simulink model "boost_cycle_R2021b"  (R2021b)
settings: Solver=FixedStepDiscrete  StartTime=0  StopTime=(N-1)*Ts  FixedStep=Ts  RelTol=1e-3
model workspace (MAT data in the model file):
  CP = [2 0.03 20 0 0 1 0 0 0.15 12 12 48 0.5 0.05 0.9 0.0005 5e-05 0 60 0 18 0 15 0 60 24 0 0 0 0 0 0]
  LP = [1 0.05 20 10 0 0 0]
  N = 2000
  PP = [0.0005 0.00047 5e-05 0 0 0 0 100 0 0]
  Ts = 5e-05
  VP = [0 24 0 0 0 0 0]
  X0 = [0; 0; 0; 0; 0; 0.5; 0.5; 0.5]
  XP0 = [0; 24; 24]
settings Model: Creator=runner  LastModifiedBy=runner
settings DebuggingCC: AlgebraicLoopMsg=error  UnconnectedInputMsg=none  UnconnectedOutputMsg=none  UnconnectedLineMsg=none
settings ModelReferenceCC: EnableRefExpFcnMdlSchedulingChecks=off
settings RTWCC: DLArmComputeVersion=20.02.1

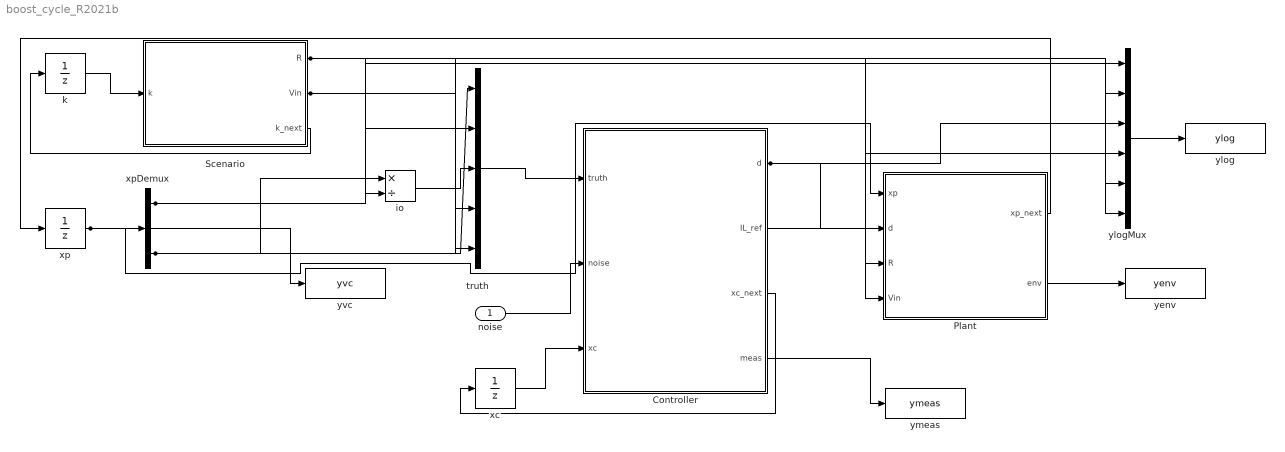
== system boost_cycle_R2021b ==
  noise : Inport  PortDimensions=4  SampleTime=Ts
  Controller : MATLAB Function  TreatAsAtomicUnit=on
  Plant : MATLAB Function  TreatAsAtomicUnit=on
  Scenario : MATLAB Function  TreatAsAtomicUnit=on
  io : Product  Inputs=*/
  k : UnitDelay  SampleTime=Ts  HasFrameUpgradeWarning=on
  truth : Mux  Inputs=5
  xc : UnitDelay  InitialCondition=X0  SampleTime=Ts  HasFrameUpgradeWarning=on
  xp : UnitDelay  InitialCondition=XP0  SampleTime=Ts  HasFrameUpgradeWarning=on
  xpDemux : Demux  Outputs=3
  yenv : ToWorkspace  VariableName=yenv  SampleTime=Ts
  ylog : ToWorkspace  VariableName=ylog  SampleTime=Ts
  ylogMux : Mux  Inputs=6
  ymeas : ToWorkspace  VariableName=ymeas  SampleTime=Ts
  yvc : ToWorkspace  VariableName=yvc  SampleTime=Ts
  wires:
  k/1 -> Scenario/1(k)
  Scenario/3(k_next) -> k/1
  xp/1 -> xpDemux/1, Plant/1(xp)
  xpDemux/3 -> io/1, truth/1, ylogMux/1
  Scenario/1(R) -> io/2, truth/5, Plant/3(R), ylogMux/5
  xpDemux/1 -> truth/2, ylogMux/2
  io/1 -> truth/3
  Scenario/2(Vin) -> truth/4, Plant/4(Vin), ylogMux/6
  truth/1 -> Controller/1(truth)
  noise/1 -> Controller/2(noise)
  xc/1 -> Controller/3(xc)
  Controller/3(xc_next) -> xc/1
  Controller/1(d) -> Plant/2(d), ylogMux/3
  Plant/1(xp_next) -> xp/1
  Controller/2(IL_ref) -> ylogMux/4
  ylogMux/1 -> ylog/1
  Controller/4(meas) -> ymeas/1
  Plant/2(env) -> yenv/1
  xpDemux/2 -> yvc/1

== matlab function boost_cycle_R2021b/Controller ==
  settings: updateMethod=DISCRETE  sampleTime=Ts
  data: truth input; d output; noise input; xc input double size=[8 1]; IL_ref output; xc_next output; meas output; CP parameter
function [d, IL_ref, xc_next, meas] = ctrl(truth, noise, xc, CP)
[d, IL_ref, xc_next, meas] = blk_controller(truth, noise, xc, CP);
end

== matlab function boost_cycle_R2021b/Scenario ==
  settings: updateMethod=DISCRETE  sampleTime=Ts
  data: k input double size=1; R output; Vin output; k_next output; LP parameter; VP parameter; Ts parameter
function [R, Vin, k_next] = scen(k, LP, VP, Ts)
[R, Vin, k_next] = blk_scenario(k, LP, VP, Ts);
end

== matlab function boost_cycle_R2021b/Plant ==
  settings: updateMethod=DISCRETE  sampleTime=Ts
  data: xp input double size=[3 1]; xp_next output; d input; R input; Vin input; env output; PP parameter
function [xp_next, env] = plant(xp, d, R, Vin, PP)
[xp_next, env] = blk_plant_switched(xp, d, R, Vin, PP);
end
